simulink model "Sim_Monitors"  (R2026b)
settings: Solver=VariableStepAuto
undefined symbols (not defined in the file or in its folder): DiscIntNeverNeededParam, P, sim_monitor_obstacles, Ts
libraries: simulink x7, dspstat3 x2, robotcorelib x1
settings Model: Creator=aomar  LastModifiedBy=aomar

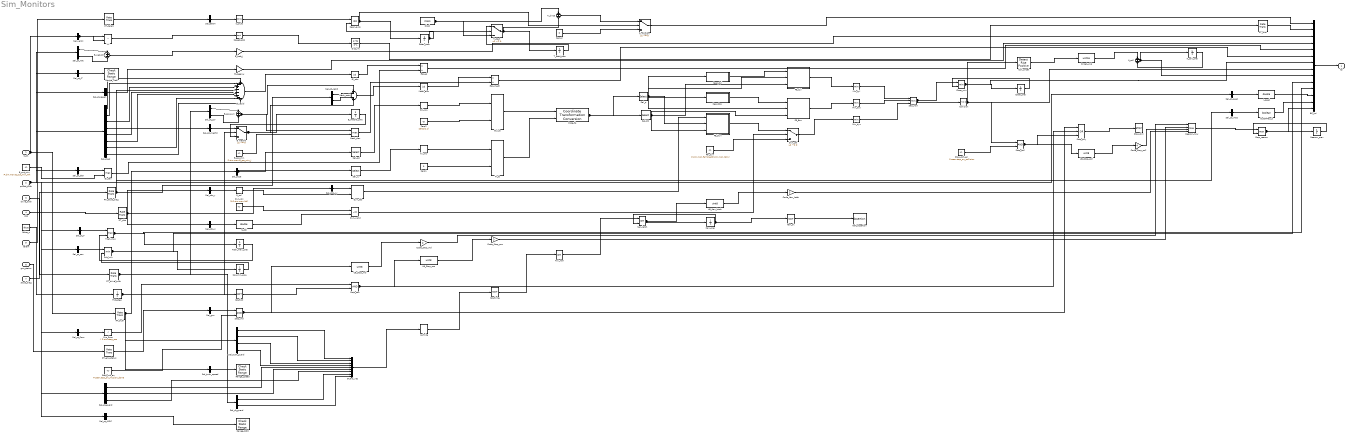
== system Sim_Monitors ==
  truth : Inport  OutDataTypeStr=Bus: Bus_TruthState  SampleTime=Ts.base
  power_truth : Inport  Port=2  OutDataTypeStr=Bus: Bus_PowerTruth  SampleTime=Ts.hk
  drive_truth : Inport  Port=3  OutDataTypeStr=Bus: Bus_DriveTruth  SampleTime=Ts.base
  obs : Inport  Port=4  OutDataTypeStr=Bus: Bus_ObstaclesDyn  SampleTime=Ts.ctrl
  telem : Inport  Port=5  OutDataTypeStr=Bus: Bus_FwTelemetry  SampleTime=Ts.ctrl
  gnc_status : Inport  Port=6  OutDataTypeStr=Bus: Bus_GncStatus  SampleTime=Ts.gnc_status
  struct_diag : Inport  Port=7  OutDataTypeStr=Bus: Bus_StructureDiag  SampleTime=Ts.ctrl
  Any_nan : Logic  Operator=OR  Inputs=1  AllPortsSameDT=off  OutDataTypeStr=boolean
  BC_kpi : BusCreator  Inputs=14  OutDataTypeStr=Bus: Bus_SimKPI  NonVirtualBus=on
  Clear_min : MinMax  Inputs=2
  Clear_prev : UnitDelay  InitialCondition=P.sim.mon.far  SampleTime=Ts.monitor
  Clock : DigitalClock  SampleTime=Ts.monitor
  Code_Nan_latch : Gain  Gain=5  ParamDataTypeStr=uint8  OutDataTypeStr=uint8
  Code_Stop_coll : Gain  Gain=4  ParamDataTypeStr=uint8  OutDataTypeStr=uint8
  Code_Stop_md : Gain  Gain=2  ParamDataTypeStr=uint8  OutDataTypeStr=uint8
  Code_Stop_soc : Gain  Gain=3  ParamDataTypeStr=uint8  OutDataTypeStr=uint8
  Coll_onset : simulink/Logic and Bit Operations/Detect Rise Positive  vinit=0  OutDataTypeStr=boolean
  Collision : simulink/Logic and Bit Operations/Compare To Zero  relop=<=  OutDataTypeStr=boolean
  Dist_int : DiscreteIntegrator  SampleTime=Ts.base  ICPrevOutput=DiscIntNeverNeededParam  ICPrevScaledInput=DiscIntNeverNeededParam
  Dyn_idx : Constant  Value=(1:P.sim.mon.Nd)'  VectorParams1D=off  SampleTime=Ts.monitor
  Dyn_sel : Switch  Criteria=u2 ~= 0  SaturateOnIntegerOverflow=off  InputSameDT=off
  Dyn_tab : Concatenate  Mode=Multidimensional array  ConcatenateDimension=2
  Dyn_valid : RelationalOperator  Operator=<=  OutDataTypeStr=boolean  RndMeth=Simplest  InputSameDT=off
  E_batt_J : Gain  Gain=3600
  E_mech0 : Switch  Criteria=u2 ~= 0  SaturateOnIntegerOverflow=off  InputSameDT=off
  E_mech0_prev : UnitDelay  SampleTime=Ts.monitor
  E_net_Wh : Sum  Inputs=+-
  E_out_min : Constant  Value=P.sim.mon.E_out_min_Wh  VectorParams1D=off  SampleTime=Ts.monitor
  E_regen_J : Gain  Gain=3600
  E_spr_min : Constant  Value=P.sim.mon.E_spr_min_J  VectorParams1D=off  SampleTime=Ts.monitor
  E_spr_sum : Sum
  El_abs : Abs  SaturateOnIntegerOverflow=off
  El_den : MinMax  Function=max  Inputs=2
  El_resid : Sum  Inputs=+-+-----
  Eps_el : Product  Inputs=*/
  Eps_mech : Product  Inputs=*/
  Eul_fp : Concatenate  Mode=Multidimensional array
  FE_Box : Subsystem  Description=Planar separation footprint <-> obstacle (rect), one iteration per table row (5 columns): MATLAB Function Sep -> mon_sep_rect (D70).  TreatAsAtomicUnit=on
  FE_Cyl : Subsystem  Description=Planar separation footprint <-> obstacle (circle), one iteration per table row (3 columns): MATLAB Function Sep -> mon_sep_circle (D70).  TreatAsAtomicUnit=on
  FE_Dyn : Subsystem  Description=Planar separation footprint <-> obstacle (circle), one iteration per table row (3 columns): MATLAB Function Sep -> mon_sep_circle (D70).  TreatAsAtomicUnit=on
  False_c : Constant  Value=false  VectorParams1D=off  OutDataTypeStr=boolean  SampleTime=Ts.monitor
  Far_dyn : Constant  Value=P.sim.mon.far*ones(P.sim.mon.Nd,1)  VectorParams1D=off  SampleTime=Ts.monitor
  First_step : UnitDelay  InitialCondition=true  SampleTime=Ts.monitor
  Guard_vec : Concatenate  NumInputs=9
  I_peak : DataTypeConversion  OutDataTypeStr=double  SaturateOnIntegerOverflow=off  RndMeth=Floor
  Is_auto : simulink/Logic and Bit Operations/Compare To Constant  relop===  const=6  OutDataTypeStr=boolean
  Is_finite : RelationalOperator  Operator=isFinite  OutDataTypeStr=boolean  RndMeth=Simplest  InputSameDT=off
  Mech_abs : Abs  SaturateOnIntegerOverflow=off
  Mech_den : MinMax  Function=max  Inputs=2
  Mech_resid : Sum  Inputs=+--+
  Min_box : MinMax
  Min_cyl : MinMax
  Min_dyn : MinMax
  N_coll : Sum  OutDataTypeStr=uint16  SaturateOnIntegerOverflow=on
  N_coll_prev : UnitDelay  InitialCondition=uint16(0)  SampleTime=Ts.monitor
  N_dbl : DataTypeConversion  OutDataTypeStr=double  SaturateOnIntegerOverflow=off  RndMeth=Floor
  NaN_Assertion : Assertion  SampleTime=Ts.monitor
  Nan_latch : Logic  Operator=OR  AllPortsSameDT=off  OutDataTypeStr=boolean
  Nan_ok : Logic  Operator=NOT  AllPortsSameDT=off  OutDataTypeStr=boolean
  Nan_prev : UnitDelay  InitialCondition=false  SampleTime=Ts.monitor
  Near_Box : Subsystem  Description=Nearest P.sim.mon.Kb rows of sim_monitor_obstacles(P.world,'box',P.sim.mon) (5 columns) to the footprint centre.
  Near_Cyl : Subsystem  Description=Nearest P.sim.mon.Kc rows of sim_monitor_obstacles(P.world,'cyl',P.sim.mon) (3 columns) to the footprint centre.
  Not_finite : Logic  Operator=NOT  AllPortsSameDT=off  OutDataTypeStr=boolean
  Not_first : Logic  Operator=NOT  AllPortsSameDT=off  OutDataTypeStr=boolean
  Onset_u16 : DataTypeConversion  OutDataTypeStr=uint16  SaturateOnIntegerOverflow=off  RndMeth=Floor
  OutOfMap_b : DataTypeConversion  OutDataTypeStr=boolean  SaturateOnIntegerOverflow=off  RndMeth=Floor
  Pose_fp : robotcorelib/Coordinate Transformation Conversion  InputRepresentation=Euler Angles  InputEulerSequence=ZYX  ShowTrVecInputPort=on  OutputRepresentation=Homogeneous Transformation  OutputEulerSequence=ZYX  ShowTrVecOutputPort=on  SimulateUsing=Interpreted execution
      settings: LibrarySourceBlock=navlib/Utilities/Coordinate Transformation Conversion
  Psi_row : Reshape  OutputDimensionality=Column vector (2-D)
  RT_dist : RateTransition  OutPortSampleTime=Ts.monitor
  RT_drive_truth : RateTransition  InitialCondition=P.ic.Bus_DriveTruth  OutPortSampleTime=Ts.monitor
  RT_gnc_status : RateTransition  InitialCondition=P.ic.Bus_GncStatus  OutPortSampleTime=Ts.monitor
  RT_obs : RateTransition  InitialCondition=P.ic.Bus_ObstaclesDyn  OutPortSampleTime=Ts.monitor
  RT_struct_diag : RateTransition  InitialCondition=P.ic.Bus_StructureDiag  OutPortSampleTime=Ts.monitor
  RT_telem : RateTransition  InitialCondition=P.ic.Bus_FwTelemetry  OutPortSampleTime=Ts.monitor
  RT_truth : RateTransition  InitialCondition=P.ic.Bus_TruthState  OutPortSampleTime=Ts.monitor
  R_col : Reshape  OutputDimensionality=Column vector (2-D)
  Range_SOC : simulink/Model Verification/Check  Static Range  Description=0 <= u <= 1  max=1  max_included=on  min=0  min_included=on  enabled=on  stopWhenAssertionFail=off  export=off  icon=graphic
  Range_Tcell : simulink/Model Verification/Check  Static Range  Description=P.sim.mon.T_cell_rng(1) <= u <= P.sim.mon.T_cell_rng(2)  max=P.sim.mon.T_cell_rng(2)  max_included=on  min=P.sim.mon.T_cell_rng(1)  min_included=on  enabled=on  stopWhenAssertionFail=off  export=off  icon=graphic
  Range_speed : simulink/Model Verification/Check  Static Range  Description=-P.sim.mon.v_abs_max <= u <= P.sim.mon.v_abs_max  max=P.sim.mon.v_abs_max  max_included=on  min=-P.sim.mon.v_abs_max  min_included=on  enabled=on  stopWhenAssertionFail=off  export=off  icon=graphic
  Reason_now : MinMax  Function=max  Inputs=4  OutDataTypeStr=uint8
  Reason_prev : UnitDelay  InitialCondition=uint8(0)  SampleTime=Ts.monitor
  Seen_auto : Logic  Operator=OR  AllPortsSameDT=off  OutDataTypeStr=boolean
  Seen_prev : UnitDelay  InitialCondition=false  SampleTime=Ts.monitor
  Sel_R2 : Selector  NumberOfDimensions=2  InputPortWidth=3  IndexOptions=Index vector (dialog),Index vector (dialog)  Indices=[1 2],[1 2]  OutputSizes=1
  Sel_dt_guard : BusSelector  OutputSignals=L.w_m,R.w_m
  Sel_dt_spr : BusSelector  OutputSignals=L.E_spr,R.E_spr
  Sel_gnc : BusSelector  OutputSignals=mission_done
  Sel_obs_n : BusSelector  OutputSignals=n
  Sel_obs_r : BusSelector  OutputSignals=r
  Sel_obs_xy : BusSelector  OutputSignals=xy
  Sel_p : Selector  NumberOfDimensions=2  InputPortWidth=3  IndexOptions=Index vector (dialog),Index vector (dialog)  Indices=[1 2],4  OutputSizes=1
  Sel_pose : BusSelector  OutputSignals=pose2D
  Sel_psi : Selector  InputPortWidth=3  IndexOptions=Index vector (dialog)  Indices=3  OutputSizes=1
  Sel_pt_T : BusSelector  OutputSignals=T_cell_max_K
  Sel_pt_den : BusSelector  OutputSignals=E_out_Wh
  Sel_pt_el : BusSelector  OutputSignals=E_out_Wh,E_in_Wh,E_chg_bus_Wh,E_trac_dc_Wh,E_impl_dc_Wh,E_lv_Wh,E_dcdc_loss_Wh,E_pdu_loss_Wh
  Sel_pt_floor : BusSelector  OutputSignals=SOC_pack_true
  Sel_pt_guard : BusSelector  OutputSignals=SOC_pack_true,I_pack_A,V_term_V
  Sel_pt_net : BusSelector  OutputSignals=E_out_Wh,E_in_Wh
  Sel_pt_peak : BusSelector  OutputSignals=I_pack_peak_A
  Sel_pt_rSOC : BusSelector  OutputSignals=SOC_pack_true
  Sel_pt_rT : BusSelector  OutputSignals=T_cell_max_K
  Sel_pt_regen : BusSelector  OutputSignals=E_in_Wh
  Sel_pt_soc : BusSelector  OutputSignals=SOC_pack_true
  Sel_sd_map : BusSelector  OutputSignals=outOfMap
  Sel_sd_mech0 : BusSelector  OutputSignals=E_mech
  Sel_sd_resid : BusSelector  OutputSignals=E_diss_J,E_mech
  Sel_telem : BusSelector  OutputSignals=mode
  Sel_truth_guard : BusSelector  OutputSignals=pos_W,vel_W,eul,omega_B
  Sel_truth_speed : BusSelector  OutputSignals=speed_fwd
  Sel_vel1k : BusSelector  OutputSignals=vel_W
  Sel_xy : Selector  InputPortWidth=3  IndexOptions=Index vector (dialog)  Indices=[1 2]  OutputSizes=1
  Sep_now : MinMax  Inputs=3
  Soc_floor : simulink/Logic and Bit Operations/Compare To Constant  relop=<  const=P.sim.stop_soc  OutDataTypeStr=boolean
  Soc_min : MinMax  Inputs=2
  Soc_min_prev : UnitDelay  InitialCondition=P.sim.mon.far  SampleTime=Ts.monitor
  Speed_abs : Sqrt
  Stop_Sim : Stop
  Stop_any : Logic  Operator=OR  Inputs=3  AllPortsSameDT=off  OutDataTypeStr=boolean
  Stop_coll : Logic  AllPortsSameDT=off  OutDataTypeStr=boolean
  Stop_coll_en : Constant  Value=P.scen.stop_on_collision  VectorParams1D=off  OutDataTypeStr=boolean  SampleTime=Ts.monitor
  Stop_md : Logic  AllPortsSameDT=off  OutDataTypeStr=boolean
  Stop_md_en : Constant  Value=P.scen.stop_on_mission_done  VectorParams1D=off  OutDataTypeStr=boolean  SampleTime=Ts.monitor
  Stop_reason : MinMax  Function=max  Inputs=2  OutDataTypeStr=uint8
  Stop_soc : Logic  AllPortsSameDT=off  OutDataTypeStr=boolean
  T_mission : Switch  Criteria=u2 ~= 0  SaturateOnIntegerOverflow=off  InputSameDT=off
  T_since : Sum  Inputs=+-
  T_start : Switch  Criteria=u2 ~= 0  SaturateOnIntegerOverflow=off  InputSameDT=off
  T_start_prev : UnitDelay  SampleTime=Ts.monitor
  Tcell_max : MinMax  Function=max  Inputs=2
  Tcell_max_prev : UnitDelay  InitialCondition=-P.sim.mon.far  SampleTime=Ts.monitor
  Tr_fp : Concatenate  Mode=Multidimensional array
  U8_Nan_latch : DataTypeConversion  OutDataTypeStr=uint8  SaturateOnIntegerOverflow=off  RndMeth=Floor
  U8_Stop_coll : DataTypeConversion  OutDataTypeStr=uint8  SaturateOnIntegerOverflow=off  RndMeth=Floor
  U8_Stop_md : DataTypeConversion  OutDataTypeStr=uint8  SaturateOnIntegerOverflow=off  RndMeth=Floor
  U8_Stop_soc : DataTypeConversion  OutDataTypeStr=uint8  SaturateOnIntegerOverflow=off  RndMeth=Floor
  VV : DotProduct  OutDataTypeStr=Inherit: Inherit via internal rule
  XY_row : Reshape  OutputDimensionality=Column vector (2-D)
  Zero1 : Constant  Value=0  VectorParams1D=off  SampleTime=Ts.monitor
  Zero2 : Constant  Value=zeros(2,1)  VectorParams1D=off  SampleTime=Ts.monitor
  Zero_t : Constant  Value=0  VectorParams1D=off  SampleTime=Ts.monitor
  kpi : Outport  OutDataTypeStr=Bus: Bus_SimKPI
  wires:
  truth/1 -> RT_truth/1, Sel_vel1k/1  "truth"
  E_out_min/1 -> El_den/2  "E_out_min"
  power_truth/1 -> Sel_pt_rSOC/1, Sel_pt_guard/1, Sel_pt_floor/1, Sel_pt_net/1, Sel_pt_rT/1, Sel_pt_regen/1, Sel_pt_peak/1, Sel_pt_soc/1, Sel_pt_el/1, Sel_pt_T/1, Sel_pt_den/1  "power_truth"
  drive_truth/1 -> RT_drive_truth/1  "drive_truth"
  obs/1 -> RT_obs/1  "obs"
  False_c/1 -> First_step/1  "False_c"
  telem/1 -> RT_telem/1  "telem"
  gnc_status/1 -> RT_gnc_status/1  "gnc_status"
  struct_diag/1 -> RT_struct_diag/1  "struct_diag"
  Sel_vel1k/1 -> VV/2, VV/1  "<vel_W>"
  Sel_pt_net/1 -> E_net_Wh/1  "<E_out_Wh>"
  Sel_pt_net/2 -> E_net_Wh/2  "<E_in_Wh>"
  Sel_pt_rT/1 -> Range_Tcell/1  "<T_cell_max_K>"
  Sel_pt_den/1 -> El_den/1  "<E_out_Wh>"
  Sel_pt_soc/1 -> Soc_min/1  "<SOC_pack_true>"
  Sel_pt_floor/1 -> Soc_floor/1  "<SOC_pack_true>"
  Sel_pt_T/1 -> Tcell_max/1  "<T_cell_max_K>"
  Sel_pt_regen/1 -> E_regen_J/1  "<E_in_Wh>"
  Sel_pt_el/1 -> El_resid/1  "<E_out_Wh>"
  Sel_pt_el/2 -> El_resid/2  "<E_in_Wh>"
  Sel_pt_el/3 -> El_resid/3  "<E_chg_bus_Wh>"
  Sel_pt_el/4 -> El_resid/4  "<E_trac_dc_Wh>"
  Sel_pt_el/5 -> El_resid/5  "<E_impl_dc_Wh>"
  Sel_pt_el/6 -> El_resid/6  "<E_lv_Wh>"
  Sel_pt_el/7 -> El_resid/7  "<E_dcdc_loss_Wh>"
  Sel_pt_el/8 -> El_resid/8  "<E_pdu_loss_Wh>"
  Sel_pt_guard/1 -> Guard_vec/5  "<SOC_pack_true>"
  Sel_pt_guard/2 -> Guard_vec/6  "<I_pack_A>"
  Sel_pt_guard/3 -> Guard_vec/7  "<V_term_V>"
  Sel_pt_rSOC/1 -> Range_SOC/1  "<SOC_pack_true>"
  E_net_Wh/1 -> E_batt_J/1  "E_net_Wh"
  VV/1 -> Speed_abs/1  "VV"
  El_den/1 -> Eps_el/2  "El_den"
  Soc_min/1 -> BC_kpi/10, Soc_min_prev/1  "soc_min"
  Soc_floor/1 -> Stop_soc/1  "Soc_floor"
  Stop_md_en/1 -> Stop_md/2  "Stop_md_en"
  RT_telem/1 -> Sel_telem/1  "telem_10Hz"
  Tcell_max/1 -> BC_kpi/11, Tcell_max_prev/1  "T_cell_max"
  RT_gnc_status/1 -> Sel_gnc/1  "gnc_status_10Hz"
  RT_struct_diag/1 -> Sel_sd_resid/1, Sel_sd_map/1, Sel_sd_mech0/1  "struct_diag_10Hz"
  First_step/1 -> E_mech0/2, Not_first/1  "first_step"
  RT_truth/1 -> Sel_pose/1, Sel_truth_speed/1, Sel_truth_guard/1  "truth_10Hz"
  Sel_telem/1 -> Is_auto/1  "<mode>"
  Sel_dt_spr/1 -> E_spr_sum/1  "<E_spr>"
  Sel_dt_spr/2 -> E_spr_sum/2  "<E_spr>"
  Sel_sd_mech0/1 -> E_mech0/1  "<E_mech>"
  Sel_obs_r/1 -> R_col/1  "<r>"
  Sel_obs_n/1 -> N_dbl/1  "<n>"
  Sel_gnc/1 -> Stop_md/1  "<mission_done>"
  Sel_truth_speed/1 -> Range_speed/1  "<speed_fwd>"
  Sel_pose/1 -> Sel_psi/1, Sel_xy/1  "<pose2D>"
  Sel_truth_guard/1 -> Guard_vec/1  "<pos_W>"
  Sel_truth_guard/2 -> Guard_vec/2  "<vel_W>"
  Sel_truth_guard/3 -> Guard_vec/3  "<eul>"
  Sel_truth_guard/4 -> Guard_vec/4  "<omega_B>"
  Sel_dt_guard/1 -> Guard_vec/8  "<w_m>"
  Sel_dt_guard/2 -> Guard_vec/9  "<w_m>"
  E_spr_sum/1 -> Mech_resid/1, Mech_den/1  "E_spr_sum"
  Is_auto/1 -> Seen_auto/1  "Is_auto"
  Speed_abs/1 -> Dist_int/1  "speed_abs"
  E_batt_J/1 -> BC_kpi/3  "E_batt"
  E_regen_J/1 -> BC_kpi/4  "E_regen"
  E_spr_min/1 -> Mech_den/2  "E_spr_min"
  R_col/1 -> Dyn_tab/2  "R_col"
  Dyn_idx/1 -> Dyn_valid/1  "Dyn_idx"
  Not_first/1 -> Stop_soc/2  "Not_first"
  Stop_md/1 -> Stop_any/1, U8_Stop_md/1  "stop_md"
  Tcell_max_prev/1 -> Tcell_max/2  "Tcell_max_prev"
  Soc_min_prev/1 -> Soc_min/2  "Soc_min_prev"
  El_resid/1 -> El_abs/1  "El_resid"
  E_mech0/1 -> Mech_resid/4, E_mech0_prev/1  "E_mech0"
  N_dbl/1 -> Dyn_valid/2  "N_dbl"
  Sel_sd_resid/1 -> Mech_resid/2  "<E_diss_J>"
  Sel_sd_resid/2 -> Mech_resid/3  "<E_mech>"
  Sel_obs_xy/1 -> Dyn_tab/1  "<xy>"
  Guard_vec/1 -> Is_finite/1  "guard_vec"
  Mech_resid/1 -> Mech_abs/1  "Mech_resid"
  Seen_auto/1 -> Seen_prev/1, T_mission/2  "seen_auto"
  El_abs/1 -> Eps_el/1  "El_abs"
  Mech_den/1 -> Eps_mech/2  "Mech_den"
  Dyn_valid/1 -> Dyn_sel/2  "dyn_valid"
  Stop_soc/1 -> Stop_any/2, U8_Stop_soc/1  "stop_soc"
  Dist_int/1 -> RT_dist/1  "Dist_int"
  E_mech0_prev/1 -> E_mech0/3  "E_mech0_prev"
  Sel_psi/1 -> Psi_row/1  "Sel_psi"
  Sel_xy/1 -> XY_row/1  "Sel_xy"
  Dyn_tab/1 -> FE_Dyn/1(row)  "dyn_tab"
  U8_Stop_md/1 -> Code_Stop_md/1  "U8_Stop_md"
  Eps_el/1 -> BC_kpi/5  "eps_el"
  Mech_abs/1 -> Eps_mech/1  "Mech_abs"
  Psi_row/1 -> Eul_fp/1  "Psi_row"
  Zero2/1 -> Eul_fp/2  "Zero2"
  XY_row/1 -> Tr_fp/1  "XY_row"
  Zero1/1 -> Tr_fp/2  "Zero1"
  Code_Stop_md/1 -> Reason_now/1  "Code_Stop_md"
  Is_finite/1 -> Not_finite/1  "Is_finite"
  Seen_prev/1 -> Seen_auto/2, T_start/2  "seen_auto_prev"
  Clock/1 -> T_start/3, T_since/1  "t"
  U8_Stop_soc/1 -> Code_Stop_soc/1  "U8_Stop_soc"
  Eps_mech/1 -> BC_kpi/6  "eps_mech"
  Code_Stop_soc/1 -> Reason_now/2  "Code_Stop_soc"
  Not_finite/1 -> Any_nan/1  "Not_finite"
  T_start/1 -> T_start_prev/1, T_since/2  "t_start"
  Eul_fp/1 -> Pose_fp/1  "eul_fp"
  Tr_fp/1 -> Pose_fp/2  "trvec_fp"
  T_since/1 -> T_mission/1  "T_since"
  Zero_t/1 -> T_mission/3  "Zero_t"
  Any_nan/1 -> Nan_latch/1  "nan_now"
  T_start_prev/1 -> T_start/1  "T_start_prev"
  Pose_fp/1 -> Sel_p/1, Sel_R2/1  "T_fp"
  Nan_latch/1 -> U8_Nan_latch/1, Nan_prev/1  "nan_latched"
  Sel_p/1 -> FE_Dyn/2(p), Near_Cyl/1(p), FE_Cyl/2(p), FE_Box/2(p), Near_Box/1(p)  "fp_p"
  T_mission/1 -> BC_kpi/1  "t_mission"
  Sel_R2/1 -> FE_Cyl/3(R), FE_Dyn/3(R), FE_Box/3(R)  "fp_R"
  Far_dyn/1 -> Dyn_sel/3  "Far_dyn"
  Nan_prev/1 -> Nan_ok/1, Nan_latch/2  "nan_prev"
  U8_Nan_latch/1 -> Code_Nan_latch/1  "U8_Nan_latch"
  Near_Cyl/1(rows) -> FE_Cyl/1(row)  "cyl_near"
  Near_Box/1(rows) -> FE_Box/1(row)  "box_near"
  FE_Dyn/1(sep) -> Dyn_sel/1  "FE_Dyn"
  Code_Nan_latch/1 -> Reason_now/4  "Code_Nan_latch"
  Nan_ok/1 -> NaN_Assertion/1  "nan_ok"
  Dyn_sel/1 -> Min_dyn/1  "sep_dyn"
  FE_Cyl/1(sep) -> Min_cyl/1  "sep_cyl"
  FE_Box/1(sep) -> Min_box/1  "sep_box"
  Min_cyl/1 -> Sep_now/1  "mon_sep_cyl"
  Min_box/1 -> Sep_now/2  "mon_sep_box"
  Min_dyn/1 -> Sep_now/3  "mon_sep_dyn"
  Sep_now/1 -> Clear_min/1, Collision/1  "sep_now"
  Clear_min/1 -> BC_kpi/7, Clear_prev/1  "clear_min"
  Stop_coll_en/1 -> Stop_coll/2  "Stop_coll_en"
  Collision/1 -> Stop_coll/1, Coll_onset/1, BC_kpi/8  "collision"
  Stop_coll/1 -> Stop_any/3, U8_Stop_coll/1  "stop_coll"
  Clear_prev/1 -> Clear_min/2  "Clear_prev"
  Coll_onset/1 -> Onset_u16/1  "Coll_onset"
  Stop_any/1 -> Stop_Sim/1  "stop_any"
  Onset_u16/1 -> N_coll/1  "Onset_u16"
  U8_Stop_coll/1 -> Code_Stop_coll/1  "U8_Stop_coll"
  N_coll/1 -> BC_kpi/9, N_coll_prev/1  "n_coll"
  Code_Stop_coll/1 -> Reason_now/3  "Code_Stop_coll"
  Reason_now/1 -> Stop_reason/1  "reason_now"
  N_coll_prev/1 -> N_coll/2  "N_coll_prev"
  Sel_pt_peak/1 -> I_peak/1  "<I_pack_peak_A>"
  Sel_sd_map/1 -> OutOfMap_b/1  "<outOfMap>"
  Stop_reason/1 -> BC_kpi/14, Reason_prev/1  "stop_reason"
  RT_dist/1 -> BC_kpi/2  "dist"
  I_peak/1 -> BC_kpi/12  "I_batt_peak"
  OutOfMap_b/1 -> BC_kpi/13  "out_of_map"
  BC_kpi/1 -> kpi/1  "kpi"
  Reason_prev/1 -> Stop_reason/2  "Reason_prev"
  RT_drive_truth/1 -> Sel_dt_spr/1, Sel_dt_guard/1  "drive_truth_10Hz"
  RT_obs/1 -> Sel_obs_xy/1, Sel_obs_r/1, Sel_obs_n/1  "obs_10Hz"

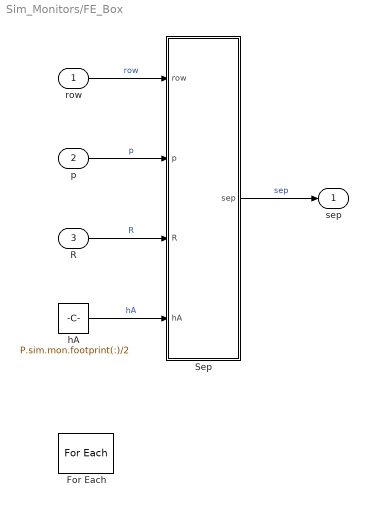
== system Sim_Monitors/FE_Box ==
  row : Inport  Partition=on  PartitionDimension=1  PartitionWidth=1  PartitionOffset=0
  p : Inport  Port=2
  R : Inport  Port=3
  For Each : ForEach  DisableCoverage=on
  Sep : MATLAB Function  TreatAsAtomicUnit=on
  hA : Constant  Value=P.sim.mon.footprint(:)/2  VectorParams1D=off  SampleTime=-1
  sep : Outport  PortDimensions=[1 1]  ConcatenationDimension=1
  wires:
  row/1 -> Sep/1(row)  "row"
  p/1 -> Sep/2(p)  "p"
  R/1 -> Sep/3(R)  "R"
  hA/1 -> Sep/4(hA)  "hA"
  Sep/1(sep) -> sep/1  "sep"

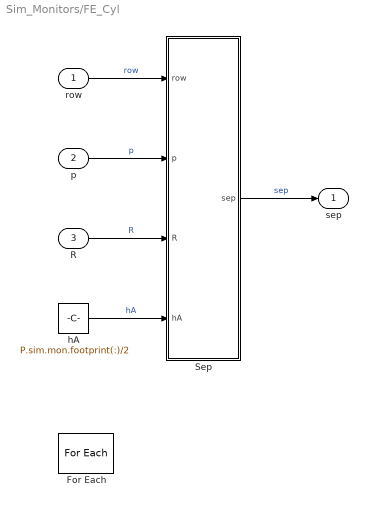
== system Sim_Monitors/FE_Cyl ==
  row : Inport  Partition=on  PartitionDimension=1  PartitionWidth=1  PartitionOffset=0
  p : Inport  Port=2
  R : Inport  Port=3
  For Each : ForEach  DisableCoverage=on
  Sep : MATLAB Function  TreatAsAtomicUnit=on
  hA : Constant  Value=P.sim.mon.footprint(:)/2  VectorParams1D=off  SampleTime=-1
  sep : Outport  PortDimensions=[1 1]  ConcatenationDimension=1
  wires:
  row/1 -> Sep/1(row)  "row"
  p/1 -> Sep/2(p)  "p"
  R/1 -> Sep/3(R)  "R"
  hA/1 -> Sep/4(hA)  "hA"
  Sep/1(sep) -> sep/1  "sep"

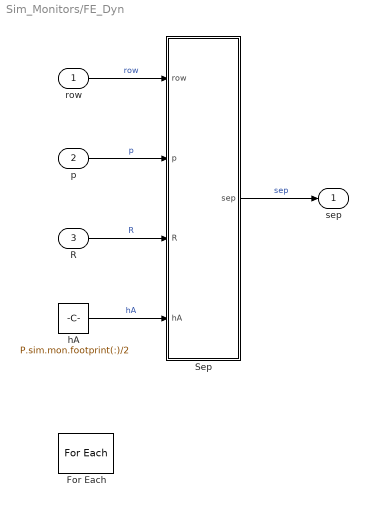
== system Sim_Monitors/FE_Dyn ==
  row : Inport  Partition=on  PartitionDimension=1  PartitionWidth=1  PartitionOffset=0
  p : Inport  Port=2
  R : Inport  Port=3
  For Each : ForEach  DisableCoverage=on
  Sep : MATLAB Function  TreatAsAtomicUnit=on
  hA : Constant  Value=P.sim.mon.footprint(:)/2  VectorParams1D=off  SampleTime=-1
  sep : Outport  PortDimensions=[1 1]  ConcatenationDimension=1
  wires:
  row/1 -> Sep/1(row)  "row"
  p/1 -> Sep/2(p)  "p"
  R/1 -> Sep/3(R)  "R"
  hA/1 -> Sep/4(hA)  "hA"
  Sep/1(sep) -> sep/1  "sep"

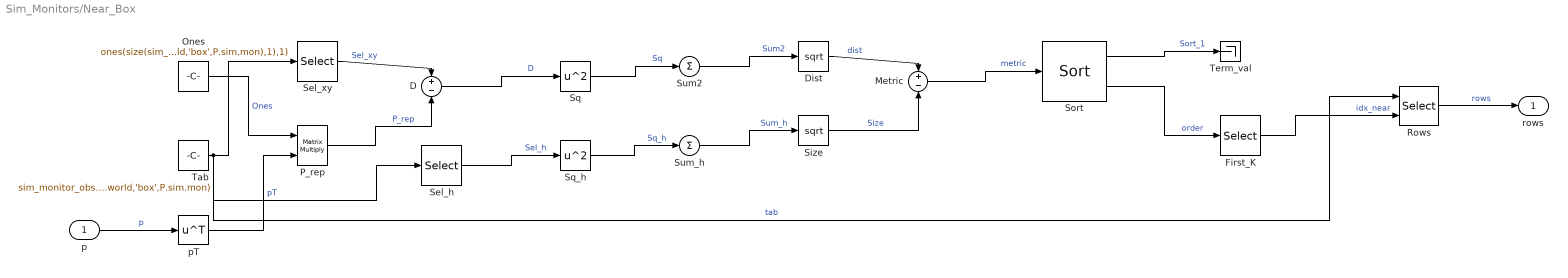
== system Sim_Monitors/Near_Box ==
  p : Inport
  D : Sum  Inputs=+-
  Dist : Sqrt
  First_K : Selector  NumberOfDimensions=2  InputPortWidth=3  IndexOptions=Starting index (dialog),Select all  Indices=1,1  OutputSizes=P.sim.mon.Kb,1
  Metric : Sum  Inputs=+-
  Ones : Constant  Value=ones(size(sim_monitor_obstacles(P.world,'box',P.sim.mon),1),1)  VectorParams1D=off  SampleTime=Ts.monitor
  P_rep : Product  Inputs=**  Multiplication=Matrix(*)
  Rows : Selector  NumberOfDimensions=2  InputPortWidth=3  IndexOptions=Index vector (port),Select all  Indices=1,1  OutputSizes=1
  Sel_h : Selector  NumberOfDimensions=2  InputPortWidth=3  IndexOptions=Select all,Index vector (dialog)  Indices=1,[4 5]  OutputSizes=1
  Sel_xy : Selector  NumberOfDimensions=2  InputPortWidth=3  IndexOptions=Select all,Index vector (dialog)  Indices=1,[1 2]  OutputSizes=1
  Size : Sqrt
  Sort : dspstat3/Sort  otype=Value and Index  dir=Ascending  sortAlg=Quick sort  roundingMode=Floor  overflowMode=off  accumDataTypeStr=Inherit: Same as product output  accumLastDataTypeStr=Inherit: Same as product output
  Sq : Math  Operator=square
  Sq_h : Math  Operator=square
  Sum2 : Sum  Inputs=+  CollapseMode=Specified dimension  CollapseDim=2
  Sum_h : Sum  Inputs=+  CollapseMode=Specified dimension  CollapseDim=2
  Tab : Constant  Value=sim_monitor_obstacles(P.world,'box',P.sim.mon)  VectorParams1D=off  SampleTime=Ts.monitor
  Term_val : Terminator
  pT : Math  Operator=transpose
  rows : Outport
  wires:
  p/1 -> pT/1  "p"
  Ones/1 -> P_rep/1  "Ones"
  Tab/1 -> Sel_xy/1, Rows/1, Sel_h/1  "tab"
  pT/1 -> P_rep/2  "pT"
  P_rep/1 -> D/2  "P_rep"
  Sel_xy/1 -> D/1  "Sel_xy"
  D/1 -> Sq/1  "D"
  Sel_h/1 -> Sq_h/1  "Sel_h"
  Sq/1 -> Sum2/1  "Sq"
  Sq_h/1 -> Sum_h/1  "Sq_h"
  Sum2/1 -> Dist/1  "Sum2"
  Sum_h/1 -> Size/1  "Sum_h"
  Dist/1 -> Metric/1  "dist"
  Size/1 -> Metric/2  "Size"
  Metric/1 -> Sort/1  "metric"
  Sort/1 -> Term_val/1  "Sort_1"
  Sort/2 -> First_K/1  "order"
  First_K/1 -> Rows/2  "idx_near"
  Rows/1 -> rows/1  "rows"

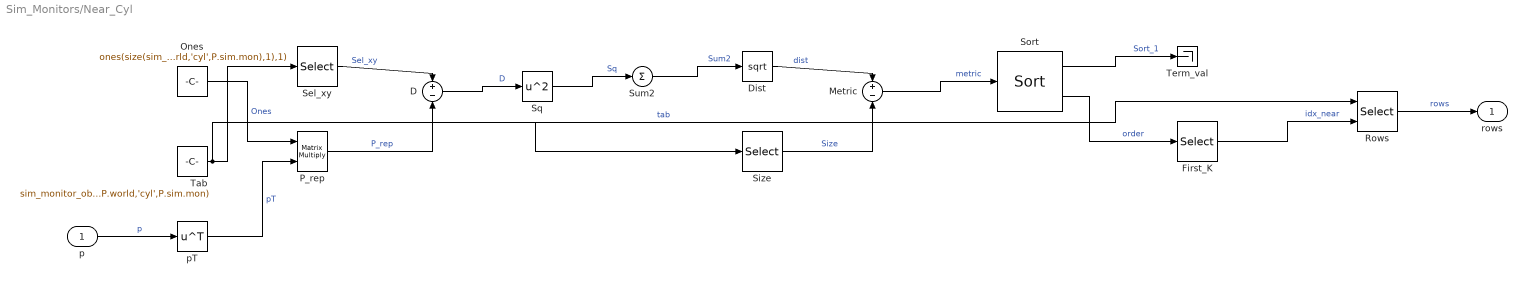
== system Sim_Monitors/Near_Cyl ==
  p : Inport
  D : Sum  Inputs=+-
  Dist : Sqrt
  First_K : Selector  NumberOfDimensions=2  InputPortWidth=3  IndexOptions=Starting index (dialog),Select all  Indices=1,1  OutputSizes=P.sim.mon.Kc,1
  Metric : Sum  Inputs=+-
  Ones : Constant  Value=ones(size(sim_monitor_obstacles(P.world,'cyl',P.sim.mon),1),1)  VectorParams1D=off  SampleTime=Ts.monitor
  P_rep : Product  Inputs=**  Multiplication=Matrix(*)
  Rows : Selector  NumberOfDimensions=2  InputPortWidth=3  IndexOptions=Index vector (port),Select all  Indices=1,1  OutputSizes=1
  Sel_xy : Selector  NumberOfDimensions=2  InputPortWidth=3  IndexOptions=Select all,Index vector (dialog)  Indices=1,[1 2]  OutputSizes=1
  Size : Selector  NumberOfDimensions=2  InputPortWidth=3  IndexOptions=Select all,Index vector (dialog)  Indices=1,3  OutputSizes=1
  Sort : dspstat3/Sort  otype=Value and Index  dir=Ascending  sortAlg=Quick sort  roundingMode=Floor  overflowMode=off  accumDataTypeStr=Inherit: Same as product output  accumLastDataTypeStr=Inherit: Same as product output
  Sq : Math  Operator=square
  Sum2 : Sum  Inputs=+  CollapseMode=Specified dimension  CollapseDim=2
  Tab : Constant  Value=sim_monitor_obstacles(P.world,'cyl',P.sim.mon)  VectorParams1D=off  SampleTime=Ts.monitor
  Term_val : Terminator
  pT : Math  Operator=transpose
  rows : Outport
  wires:
  p/1 -> pT/1  "p"
  Ones/1 -> P_rep/1  "Ones"
  Tab/1 -> Sel_xy/1, Rows/1, Size/1  "tab"
  pT/1 -> P_rep/2  "pT"
  P_rep/1 -> D/2  "P_rep"
  Sel_xy/1 -> D/1  "Sel_xy"
  D/1 -> Sq/1  "D"
  Sq/1 -> Sum2/1  "Sq"
  Sum2/1 -> Dist/1  "Sum2"
  Dist/1 -> Metric/1  "dist"
  Size/1 -> Metric/2  "Size"
  Metric/1 -> Sort/1  "metric"
  Sort/1 -> Term_val/1  "Sort_1"
  Sort/2 -> First_K/1  "order"
  First_K/1 -> Rows/2  "idx_near"
  Rows/1 -> rows/1  "rows"

== matlab function Sim_Monitors/FE_Box/Sep ==
  settings: description=Separation footprint <-> obstacle row (rect): subsystems/integration/mon_sep_rect.m (D70)
  data: row input; sep output; p input; R input; hA input
function sep = fcn(row, p, R, hA)
%#codegen
sep = mon_sep_rect(row, p, R, hA);
end

% ---- verbatim copy of subsystems/integration/mon_sep_rect.m (generated by build_sim_monitors, do not edit here) ----
function sep = mon_sep_rect(row, p, R, hA)
%MON_SEP_RECT  Separation of the robot footprint from one oriented box obstacle (Sim_Monitors FE_Box).
%
%   sep = mon_sep_rect(row, p, R, hA)
%     row  obstacle row [x y yaw hx hy] (1 x 5; world frame, m and rad; hx, hy the half extents)
%     p    footprint centre (2 x 1; world frame, m)
%     R    footprint rotation, body to world (2 x 2)
%     hA   footprint half extents (2 x 1, m): P.sim.mon.footprint(:)/2
%     sep  planar separation (m), negative when they overlap. Apart: the distance between the two rectangles,
%          the smallest signed distance of a corner of either one to the other. Overlapping (every margin of
%          the separating-axis test >= 0): minus the smallest margin, the penetration.
%
%   The MATLAB Function Sep of the For Each Subsystem FE_Box calls it once per obstacle row (D70). It does
%   what the block network did, operation for operation and in the same order, so the result is bit-identical
%   (tests/integration/t_mf_equiv, testMonitorsEquivalent). The comments name the blocks of that network.
%
%   See also mon_sep_circle, build_sim_monitors.

%#codegen
Rt = R.';                                   % Rt: world to body
d = Rt * ([row(1); row(2)] - p);            % box centre in the body frame: Sel_c, cT, Dw, d
hB = [row(4); row(5)];                      % Sel_h, hT
c = cos(row(3));                            % Sel_yaw, Cos
s = sin(row(3));                            % Sin
Rrel = Rt * [c, -s; s, c];                  % box to body: NSin, Rb_vec, Rb, Rrel
RrelT = Rrel.';                             % RrelT
one4 = ones(1, 4);                          % Ones4
S = [1 1 -1 -1; 1 -1 -1 1];                 % S, the corner signs
hA4 = hA*one4;                              % hA4
hB4 = hB*one4;                              % hB4
d4 = d*one4;                                % D4
VB = Rrel*(hB4.*S) + d4;                    % box corners in the body frame: VBloc, VBrot, VB
W = RrelT*(hA4.*S - d4);                    % footprint corners in the box frame: VAloc, VAd, W
dist = min(local_dist(VB, hA4), local_dist(W, hB4));    % BinA_*, AinB_*, Dist_min
absR = abs(Rrel);                           % AbsR
margA = hA + absR*hB - abs(d);              % on the footprint's axes: Proj_A, AbsD, Marg_A
margB = absR.'*hA + hB - abs(RrelT*d);      % on the box's axes: AbsRT, Proj_B, dB, AbsdB, Marg_B
pen = min([margA; margB]);                  % Marg, Pen
if pen >= 0                                 % Overlap
    sep = -pen;                             % NegPen
else
    sep = dist;                             % Sep (Switch)
end
end

function dist = local_dist(v, h)
% smallest signed distance of the points v (2 x 4) to the centred axis-aligned rectangle of half extents h
% (2 x 4): outside |max(q, 0)|, inside min(max(q1, q2), 0), q = |v| - h (the block group <tag>_*)
q = abs(v) - h;                             % _abs, _q
dist = min(sqrt(sum(max(q, 0).^2, 1)) + min(max(q(1, :), q(2, :)), 0));    % _qpos ... _signed, _dist
end

== matlab function Sim_Monitors/FE_Cyl/Sep ==
  settings: description=Separation footprint <-> obstacle row (circle): subsystems/integration/mon_sep_circle.m (D70)
  data: row input; sep output; p input; R input; hA input
function sep = fcn(row, p, R, hA)
%#codegen
sep = mon_sep_circle(row, p, R, hA);
end

% ---- verbatim copy of subsystems/integration/mon_sep_circle.m (generated by build_sim_monitors, do not edit here) ----
function sep = mon_sep_circle(row, p, R, hA)
%MON_SEP_CIRCLE  Separation of the robot footprint from one circular obstacle (Sim_Monitors FE_Cyl, FE_Dyn).
%
%   sep = mon_sep_circle(row, p, R, hA)
%     row  obstacle row [x y r] (1 x 3; world frame, m; r the radius)
%     p    footprint centre (2 x 1; world frame, m)
%     R    footprint rotation, body to world (2 x 2)
%     hA   footprint half extents (2 x 1, m): P.sim.mon.footprint(:)/2
%     sep  planar separation (m), negative when they overlap: the signed distance of the circle centre to the
%          footprint rectangle (outside, the distance to it; inside, minus the distance to its nearest edge),
%          minus r
%
%   The MATLAB Function Sep of the For Each Subsystems FE_Cyl and FE_Dyn calls it once per obstacle row
%   (D70). It does what their block network did, operation for operation and in the same order, so the
%   result is bit-identical (tests/integration/t_mf_equiv, testMonitorsEquivalent). The comments name the
%   blocks of that network.
%
%   See also mon_sep_rect, build_sim_monitors.

%#codegen
d = R.' * ([row(1); row(2)] - p);           % centre in the body frame: Sel_c, cT, Rt, Dw, d
q = abs(d) - hA;                            % Pt_abs, Pt_q
outside = sqrt(sum(max(q, 0).^2, 1));       % Pt_qpos, Pt_sq, Pt_sum, Pt_out
inside = min(max(q(1, :), q(2, :)), 0);     % Pt_q1, Pt_q2, Pt_qmax, Pt_in
sep = min(outside + inside) - row(3);       % Pt_signed, Pt_dist, Sel_r, Sep
end

== matlab function Sim_Monitors/FE_Dyn/Sep ==
  settings: description=Separation footprint <-> obstacle row (circle): subsystems/integration/mon_sep_circle.m (D70)
  data: row input; sep output; p input; R input; hA input
function sep = fcn(row, p, R, hA)
%#codegen
sep = mon_sep_circle(row, p, R, hA);
end

% ---- verbatim copy of subsystems/integration/mon_sep_circle.m (generated by build_sim_monitors, do not edit here) ----
function sep = mon_sep_circle(row, p, R, hA)
%MON_SEP_CIRCLE  Separation of the robot footprint from one circular obstacle (Sim_Monitors FE_Cyl, FE_Dyn).
%
%   sep = mon_sep_circle(row, p, R, hA)
%     row  obstacle row [x y r] (1 x 3; world frame, m; r the radius)
%     p    footprint centre (2 x 1; world frame, m)
%     R    footprint rotation, body to world (2 x 2)
%     hA   footprint half extents (2 x 1, m): P.sim.mon.footprint(:)/2
%     sep  planar separation (m), negative when they overlap: the signed distance of the circle centre to the
%          footprint rectangle (outside, the distance to it; inside, minus the distance to its nearest edge),
%          minus r
%
%   The MATLAB Function Sep of the For Each Subsystems FE_Cyl and FE_Dyn calls it once per obstacle row
%   (D70). It does what their block network did, operation for operation and in the same order, so the
%   result is bit-identical (tests/integration/t_mf_equiv, testMonitorsEquivalent). The comments name the
%   blocks of that network.
%
%   See also mon_sep_rect, build_sim_monitors.

%#codegen
d = R.' * ([row(1); row(2)] - p);           % centre in the body frame: Sel_c, cT, Rt, Dw, d
q = abs(d) - hA;                            % Pt_abs, Pt_q
outside = sqrt(sum(max(q, 0).^2, 1));       % Pt_qpos, Pt_sq, Pt_sum, Pt_out
inside = min(max(q(1, :), q(2, :)), 0);     % Pt_q1, Pt_q2, Pt_qmax, Pt_in
sep = min(outside + inside) - row(3);       % Pt_signed, Pt_dist, Sel_r, Sep
end
